simulink model "UAM_Hexa_PD_Obs_QGround"  (R2026a)
settings: Solver=ode4  StopTime=tf  FixedStep=0.01  EnableMultiTasking=on
values from neighbouring files (symbols this model uses):
  ArmConstants = struct('l1_dim', l1_dim,                        'l2_dim', l2_dim,                        'Hexa_to_joint_L', L,                        'Mass1', ml1,                        'Mass2', ml2,                        'Inertia1', Hl1,                        'Inertia2', Hl2,                        'MC1', c1,                        'MC2', c2,                        'Servos', Servos)    [init_model.m]    (also in init_var.m)
  HexaConstants = struct('Mass', mb,                         'Inertia', J ,                         'allo', allo,                          'invallo', invallo,                         'kT', kT)    [init_model.m]    (also in init_var.m)
  Observer = struct('E1', E1 ,     'E2', E2 ,     'E3', E3 ,     'E4', E4 ,     'MU1', MU1 ,     'MU2', MU2 ,     'MU3', MU3 ,     'alpha', alpha ,     'beta', beta)    [init_model.m]    (also in init_var.m)
libraries: px4Utilslib x189
(part 1 of 2)
settings Model: ExtModeTrigDuration=10  Creator=Carlos Fabian  LastModifiedBy=Carlos Fabian
settings SolverCC: PositivePriorityOrder=on
settings HardwareCC: ProdLargestAtomicInteger=Long  ProdLargestAtomicFloat=Double  ProdHWDeviceType=ARM Compatible->ARM Cortex
settings SFSimCC: SimTargetLang=C++
settings RTWCC: SystemTargetFile=ert.tlc  HardwareBoard=PX4 Pixhawk 6c  TLCOptions="-aInlineSetEventsForThisBaseRateFcn=TLC_FALSE -aSuppressMultiTaskScheduler=TLC_FALSE  -aRateBasedStepFcn=0"  Toolchain=GNU Tools for PX4 Autopilots  TargetLang=C++  Description=Embedded Coder
settings ERTTargetCC: ExtModeTransport=3.0  ExtModeStaticAllocSize=1024.0  SupportContinuousTime=on
settings ExplorerConfigSet: InternalSimMechanicsExplorerSettings=|
  | <ExplorerConfiguration>
  | 
  |   <canonicalview>default</canonicalview>
  | 
  |   <TilePanel>
  |     <TileInfo>
  |       <Tiles Columns="1" Count="1" Height="513" Rows="1" Width="774">
  |         <Row Weight="1"/>
  |         <Column Weight="1"/>
  |         <Tile Height="1" Width="1" X="0" Y="0"/>
  |       </Tiles>
  |     </TileInfo>
  |     <SceneInfo>
  |       <SceneViewer>
  |         <IsThisViewStd>
  |           <IsStandardView>off</IsStandardView>
  |           <StandardViewName>Front</StandardViewName>
  |         </IsThisViewStd>
  |         <BGColor>
  |           <R>1</R>
  |           <G>1</G>
  |           <B>1</B>
  |           <A>1</A>
  |         </BGColor>
  |         <Camera>
  |           <DoPerspective>off</DoPerspective>
  |           <Position>
  |             <X>16.201091586104312</X>
  |             <Y>-16.65504514146788</Y>
  |             <Z>17.087073385082522</Z>
  |           </Position>
  |           <Center>
  |             <X>-0.25720946651222221</X>
  |             <Y>-0.19674408885134653</Y>
  |             <Z>0.62877233246599318</Z>
  |           </Center>
  |           <Up>
  |             <X>-0.40824829046386302</X>
  |             <Y>0.40824829046386302</Y>
  |             <Z>0.81649658092772615</Z>
  |           </Up>
  |           <XLim>2.5491252053936631</XLim>
  |           <YLim>2.5491252053936631</YLim>
  |           <ViewLimDist>0.01</ViewLimDist>
  |         </Camera>
  |       </SceneViewer>
  |     </SceneInfo>
  |   </TilePanel>
  | 
  |   <MechEditorPanel>
  |     <GfxPanelCameraMap/>
  |     <Cameras/>
  |     <VideoCreator>
  |       <IncludeTiles>All</IncludeTiles>
  |       <IncludeTime>on</IncludeTime>
  |       <IncludeWorldFrame>off</IncludeWorldFrame>
  |       <PlaybackSpeedRatio>8</PlaybackSpeedRatio>
  |       <FrameRate>24</FrameRate>
  |       <FrameSize>auto</FrameSize>
  |       <VideoFormat>MotionJPEGAVI</VideoFormat>
  |     </VideoCreator>
  |   </MechEditorPanel>
  | 
  |   <PlaybackSettings>
  |     <PlaybackSpeedFactor>16</PlaybackSpeedFactor>
  |   </PlaybackSettings>
  | 
  | </ExplorerConfiguration>

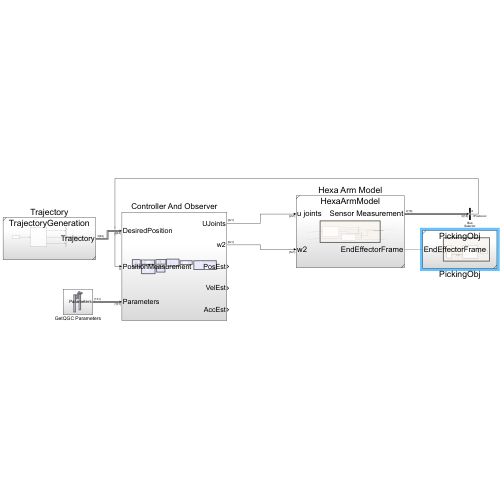
[thumbnail: Simulink's stored preview of the top-level diagram]
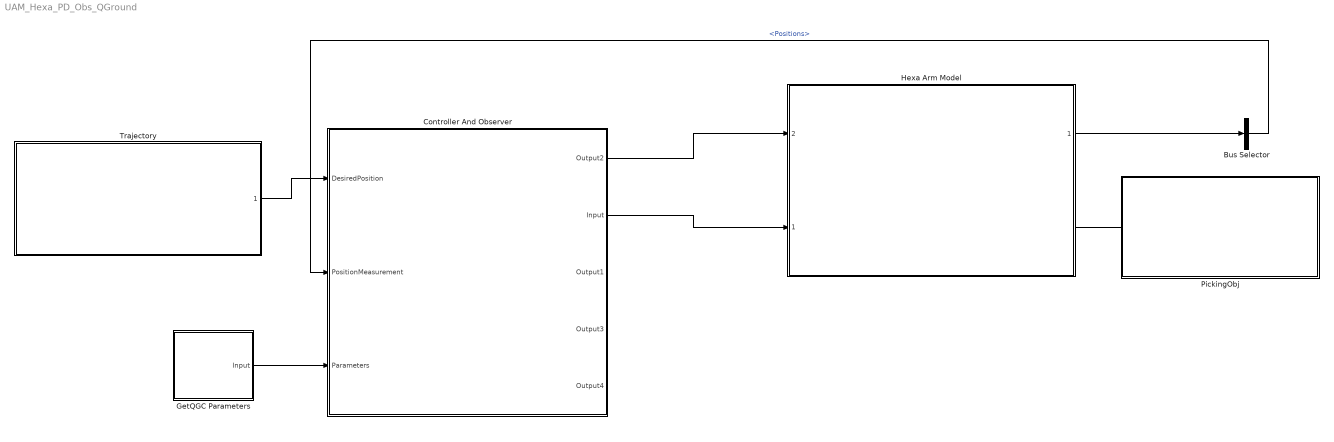
== system UAM_Hexa_PD_Obs_QGround ==
  Bus Selector : BusSelector  OutputSignals=Positions
  Controller And Observer : Subsystem
  GetQGC Parameters : Subsystem
  Hexa Arm Model : Subsystem  ReferencedSubsystem=HexaArmModel
      settings: PortSchema="{\"entries\":[{\"content\":{\"sides\":[{\"content\":{\"connectorIds\":[\"In2\",\"In1\"]},\"type\":\"ConnectorPlacement.EquallySpacedRectSide\",\"uuid\":\"8c321911-c61a-4c60-b031-eeaf4c8b5083\"},{\"content\":{\"connectorIds\":[\"Out1\",\"RConn1\"],\"side\":\"RIGHT\"},\"type\":\"ConnectorPlacement.EquallySpacedRectSide\",\"uuid\":\"3ad1588f-e2f8-4666-8b86-318f5207193d\"},{\"content\":{\"side\":\"TOP\"},\"type\":\"ConnectorPlacement.EquallySpacedRectSide\",\"uuid\":\"710cc49c-59c4-4f69-a558-4588d1d119c0\"}]},\"type\":\"ConnectorPlacement.EquallySpacedConnector\",\"uuid\":\"3e8cca1f-f7f1-4f31-9eba-ef93ff8e81e8\"}],\"packageUris\":[\"http://schema.mathworks.com/mf0/Connector/R2020b\"],\"version\":\"1.0\"}"
  PickingObj : Subsystem  ReferencedSubsystem=PickingObj
  Trajectory : Subsystem  ReferencedSubsystem=TrajectoryGeneration
  wires:
  Controller And Observer/2(Input) -> Hexa Arm Model/1
  Trajectory/1 -> Controller And Observer/1(DesiredPosition)
  Hexa Arm Model/1 -> Bus Selector/1
  Controller And Observer/1(Output2) -> Hexa Arm Model/2
  Bus Selector/1 -> Controller And Observer/2(PositionMeasurement)  "<Positions>"
  GetQGC Parameters/1(Input) -> Controller And Observer/3(Parameters)
  connections:
  Hexa Arm Model/RConn1 -- PickingObj/LConn1

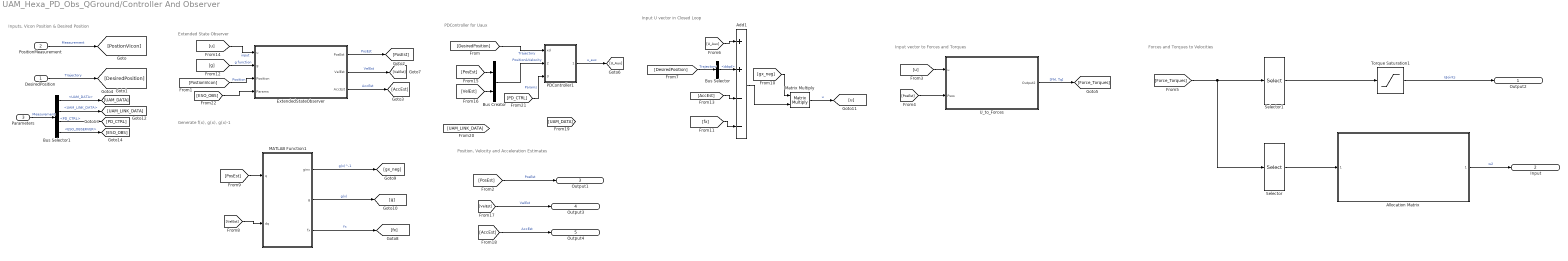
== system UAM_Hexa_PD_Obs_QGround/Controller And Observer ==
  note: Position, Velocity and Acceleration Estimates
  note: Input vector to Forces and Torques
  note: Forces and Torques to Velocities
  note: Extended State Observer
  note: Input U vector in Closed Loop
  note: Generate f(x), g(x), g(x)-1
  note: PDController for Uaux
  note: Inputs, Vicon Position & Desired Position
  DesiredPosition : Inport  SampleTime=0.01
  PositionMeasurement : Inport  Port=2  SampleTime=0.01
  Parameters : Inport  Port=3  SampleTime=0.01
  Add1 : Sum  Inputs=++--
  Allocation Matrix : Subsystem  ReferencedSubsystem=FromFMtoOmega2
  Bus Creator : BusCreator  Inputs=2
  Bus Selector : BusSelector  OutputSignals=ddqd
  Bus Selector1 : BusSelector  OutputSignals=UAM_DATA,UAM_LINK_DATA,PD_CTRL,ESO_OBSERVER
  ExtendedStateObserver : Subsystem
  MATLAB Function1 : MATLAB Function  TreatAsAtomicUnit=on
  Matrix Multiply : Product  Multiplication=Matrix(*)
  PDController1 : Subsystem
  Selector : Selector  InputPortWidth=8  IndexOptions=Index vector (dialog)  Indices=1:6  OutputSizes=1
  Selector1 : Selector  InputPortWidth=8  IndexOptions=Index vector (dialog)  Indices=7:8  OutputSizes=1
  Torque Saturation1 : Saturate  UpperLimit=ArmConstants.Servos.T1max  LowerLimit=-ArmConstants.Servos.T1max
  U_to_Forces : Subsystem
  Output2 : Outport  SampleTime=0.01
  Input : Outport  Port=2  SampleTime=0.01
  Output1 : Outport  Port=3  SampleTime=0.01
  Output3 : Outport  Port=4  SampleTime=0.01
  Output4 : Outport  Port=5  SampleTime=0.01
  wires:
  [PostionVicon] -> ExtendedStateObserver/3(Position)  "Position"
  [DesiredPosition] -> PDController1/1(xd)  "Trajectory"
  U_to_Forces/1(Output2) -> [Force_Torques]  "[FM, Tq]"
  ExtendedStateObserver/1(PosEst) -> [PosEst]  "PosEst"
  PositionMeasurement/1 -> [PostionVicon]  "Measurement"
  DesiredPosition/1 -> [DesiredPosition]  "Trajectory"
  Bus Creator/1 -> PDController1/2(q_hat1)  "Position&Velocity"
  ExtendedStateObserver/3(AccEst) -> [AccEst]  "AccEst"
  ExtendedStateObserver/2(VelEst) -> [VelEst]  "VelEst"
  [PosEst] -> U_to_Forces/2(Psos)
  Selector1/1 -> Torque Saturation1/1
  [Force_Torques] -> Selector/1, Selector1/1
  Selector/1 -> Allocation Matrix/1
  Torque Saturation1/1 -> Output2/1  "UJoints"
  Allocation Matrix/1 -> Input/1  "w2"
  PDController1/1(Output) -> [U_Aux]  "u_aux"
  MATLAB Function1/1(ginv) -> [gx_neg]  "g(x)^-1"
  MATLAB Function1/3(fx) -> [fx]  "fx"
  [VelEst] -> MATLAB Function1/2(dq)
  [PosEst] -> MATLAB Function1/1(q)
  [fx] -> Add1/4
  Add1/1 -> Matrix Multiply/2
  Matrix Multiply/1 -> [u]  "u"
  [gx_neg] -> Matrix Multiply/1
  [U_Aux] -> Add1/1
  [DesiredPosition] -> Bus Selector/1  "Trajectory"
  Bus Selector/1 -> Add1/2  "<ddqd>"
  [AccEst] -> Add1/3
  MATLAB Function1/2(g) -> [g]  "g(x)"
  [g] -> ExtendedStateObserver/2(g)  "g function"
  [u] -> ExtendedStateObserver/1(u)  "input"
  [PosEst] -> Bus Creator/1
  [VelEst] -> Bus Creator/2
  [u] -> U_to_Forces/1(u)
  [PosEst] -> Output1/1  "PosEst"
  [VelEst] -> Output3/1  "VelEst"
  [AccEst] -> Output4/1  "AccEst"
  Parameters/1 -> Bus Selector1/1  "Measurement"
  Bus Selector1/1 -> [UAM_DATA]  "<UAM_DATA>"
  Bus Selector1/4 -> [ESO_OBS]  "<ESO_OBSERVER>"
  Bus Selector1/3 -> [PD_CTRL]  "<PD_CTRL>"
  Bus Selector1/2 -> [UAM_LINK_DATA]  "<UAM_LINK_DATA>"
  [ESO_OBS] -> ExtendedStateObserver/4(Params)
  [PD_CTRL] -> PDController1/3(Params)  "Params"

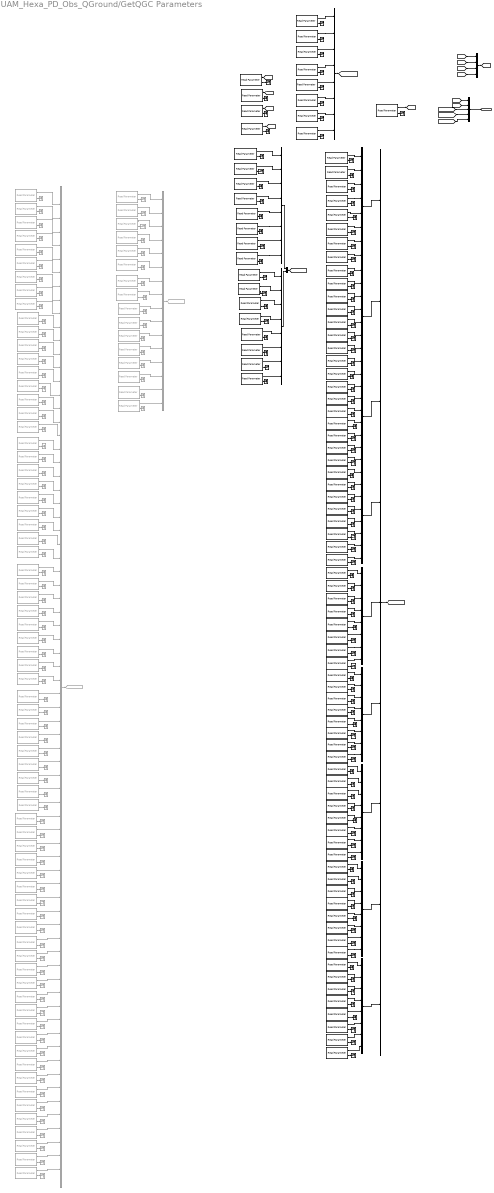
== system UAM_Hexa_PD_Obs_QGround/GetQGC Parameters ==
  note: Create Parameters Bus
  note: Parameter Manipulator
  note: Parameters FAH
  note: Parameter PD controller
  note: Parameter ESO
  note: Parameter Manipulator
  note: Parameter PD controller
  note: Parameter ESO
  Bus Creator : BusCreator  Inputs=5
  Bus Creator1 : BusCreator  Inputs=4
  Bus Creator2 : BusCreator  Inputs=2
  Bus Creator3 : BusCreator  Inputs=8
  Bus Creator4 : BusCreator  Inputs=9
  Bus Creator5 : BusCreator  Commented=on  Inputs=16
  Bus Creator6 : BusCreator  Commented=on  Inputs=72
  Goto10 : Goto  Commented=on  GotoTag=ESO_OBSERVER
  Goto9 : Goto  Commented=on  GotoTag=PD_CTRL
  Mux{,1..10} (11 alike) : Mux  Inputs=8
  Read Parameter1 : px4Utilslib/Read Parameter  ParameterName=UAM_MASS  DataType=FLOAT  SampleTime=inf
  Read Parameter10 : px4Utilslib/Read Parameter  ParameterName=UAM_L_ONE_I_ZZ  DataType=FLOAT  SampleTime=inf
  Read Parameter100 : px4Utilslib/Read Parameter  ParameterName=L_TWO_E1  DataType=FLOAT  SampleTime=inf
  Read Parameter101 : px4Utilslib/Read Parameter  ParameterName=TRAJ_SEL  DataType=INT32  SampleTime=inf
  Read Parameter102 : px4Utilslib/Read Parameter  Commented=on  ParameterName=UAM_X_P  DataType=FLOAT  SampleTime=inf
  Read Parameter103 : px4Utilslib/Read Parameter  Commented=on  ParameterName=UAM_Y_P  DataType=FLOAT  SampleTime=inf
  Read Parameter104 : px4Utilslib/Read Parameter  Commented=on  ParameterName=UAM_Y_D  DataType=FLOAT  SampleTime=inf
  Read Parameter105 : px4Utilslib/Read Parameter  Commented=on  ParameterName=UAM_Z_P  DataType=FLOAT  SampleTime=inf
  Read Parameter106 : px4Utilslib/Read Parameter  Commented=on  ParameterName=UAM_Z_D  DataType=FLOAT  SampleTime=inf
  Read Parameter107 : px4Utilslib/Read Parameter  Commented=on  ParameterName=UAM_ROLL_P  DataType=FLOAT  SampleTime=inf
  Read Parameter108 : px4Utilslib/Read Parameter  Commented=on  ParameterName=UAM_PITCH_P  DataType=FLOAT  SampleTime=inf
  Read Parameter109 : px4Utilslib/Read Parameter  Commented=on  ParameterName=UAM_PITCH_D  DataType=FLOAT  SampleTime=inf
  Read Parameter11 : px4Utilslib/Read Parameter  ParameterName=UAM_L_TWO_I_ZZ  DataType=FLOAT  SampleTime=inf
  Read Parameter110 : px4Utilslib/Read Parameter  Commented=on  ParameterName=UAM_YAW_P  DataType=FLOAT  SampleTime=inf
  Read Parameter111 : px4Utilslib/Read Parameter  Commented=on  ParameterName=UAM_YAW_D  DataType=FLOAT  SampleTime=inf
  Read Parameter112 : px4Utilslib/Read Parameter  Commented=on  ParameterName=UAM_ROLL_D  DataType=FLOAT  SampleTime=inf
  Read Parameter113 : px4Utilslib/Read Parameter  Commented=on  ParameterName=UAM_L_ONE_P  DataType=FLOAT  SampleTime=inf
  Read Parameter114 : px4Utilslib/Read Parameter  Commented=on  ParameterName=UAM_L_ONE_D  DataType=FLOAT  SampleTime=inf
  Read Parameter115 : px4Utilslib/Read Parameter  Commented=on  ParameterName=UAM_L_TWO_P  DataType=FLOAT  SampleTime=inf
  Read Parameter116 : px4Utilslib/Read Parameter  Commented=on  ParameterName=UAM_L_TWO_D  DataType=FLOAT  SampleTime=inf
  Read Parameter117 : px4Utilslib/Read Parameter  Commented=on  ParameterName=UAM_X_D  DataType=FLOAT  SampleTime=inf
  Read Parameter118 : px4Utilslib/Read Parameter  Commented=on  ParameterName=L_TWO_E1  DataType=FLOAT  SampleTime=inf
  Read Parameter119 : px4Utilslib/Read Parameter  Commented=on  ParameterName=X_E2  DataType=FLOAT  SampleTime=inf
  Read Parameter12 : px4Utilslib/Read Parameter  ParameterName=UAM_L_TWO_MASS  DataType=FLOAT  SampleTime=inf
  Read Parameter120 : px4Utilslib/Read Parameter  Commented=on  ParameterName=X_E3  DataType=FLOAT  SampleTime=inf
  Read Parameter121 : px4Utilslib/Read Parameter  Commented=on  ParameterName=X_E4  DataType=FLOAT  SampleTime=inf
  Read Parameter122 : px4Utilslib/Read Parameter  Commented=on  ParameterName=X_MU2  DataType=FLOAT  SampleTime=inf
  Read Parameter123 : px4Utilslib/Read Parameter  Commented=on  ParameterName=X_MU3  DataType=FLOAT  SampleTime=inf
  Read Parameter124 : px4Utilslib/Read Parameter  Commented=on  ParameterName=X_MU1  DataType=FLOAT  SampleTime=inf
  Read Parameter125 : px4Utilslib/Read Parameter  Commented=on  ParameterName=X_BETA  DataType=FLOAT  SampleTime=inf
  Read Parameter126 : px4Utilslib/Read Parameter  Commented=on  ParameterName=X_ALPHA  DataType=FLOAT  SampleTime=inf
  Read Parameter127 : px4Utilslib/Read Parameter  Commented=on  ParameterName=Y_E2  DataType=FLOAT  SampleTime=inf
  Read Parameter128 : px4Utilslib/Read Parameter  Commented=on  ParameterName=Y_E3  DataType=FLOAT  SampleTime=inf
  Read Parameter129 : px4Utilslib/Read Parameter  Commented=on  ParameterName=X_E1  DataType=FLOAT  SampleTime=inf
  Read Parameter13 : px4Utilslib/Read Parameter  ParameterName=UAM_L_TWO_I_XX  DataType=FLOAT  SampleTime=inf
  Read Parameter130 : px4Utilslib/Read Parameter  Commented=on  ParameterName=Y_E4  DataType=FLOAT  SampleTime=inf
  Read Parameter131 : px4Utilslib/Read Parameter  Commented=on  ParameterName=Y_MU2  DataType=FLOAT  SampleTime=inf
  Read Parameter132 : px4Utilslib/Read Parameter  Commented=on  ParameterName=Y_MU3  DataType=FLOAT  SampleTime=inf
  Read Parameter133 : px4Utilslib/Read Parameter  Commented=on  ParameterName=Y_MU1  DataType=FLOAT  SampleTime=inf
  Read Parameter134 : px4Utilslib/Read Parameter  Commented=on  ParameterName=Y_BETA  DataType=FLOAT  SampleTime=inf
  Read Parameter135 : px4Utilslib/Read Parameter  Commented=on  ParameterName=Y_ALPHA  DataType=FLOAT  SampleTime=inf
  Read Parameter136 : px4Utilslib/Read Parameter  Commented=on  ParameterName=Y_E1  DataType=FLOAT  SampleTime=inf
  Read Parameter137 : px4Utilslib/Read Parameter  Commented=on  ParameterName=Z_E2  DataType=FLOAT  SampleTime=inf
  Read Parameter138 : px4Utilslib/Read Parameter  Commented=on  ParameterName=Z_E3  DataType=FLOAT  SampleTime=inf
  Read Parameter139 : px4Utilslib/Read Parameter  Commented=on  ParameterName=Z_E4  DataType=FLOAT  SampleTime=inf
  Read Parameter14 : px4Utilslib/Read Parameter  ParameterName=UAM_L_TWO_I_YY  DataType=FLOAT  SampleTime=inf
  Read Parameter140 : px4Utilslib/Read Parameter  Commented=on  ParameterName=Z_MU2  DataType=FLOAT  SampleTime=inf
  Read Parameter141 : px4Utilslib/Read Parameter  Commented=on  ParameterName=Z_MU3  DataType=FLOAT  SampleTime=inf
  Read Parameter142 : px4Utilslib/Read Parameter  Commented=on  ParameterName=Z_MU1  DataType=FLOAT  SampleTime=inf
  Read Parameter143 : px4Utilslib/Read Parameter  Commented=on  ParameterName=Z_BETA  DataType=FLOAT  SampleTime=inf
  Read Parameter144 : px4Utilslib/Read Parameter  Commented=on  ParameterName=Z_ALPHA  DataType=FLOAT  SampleTime=inf
  Read Parameter145 : px4Utilslib/Read Parameter  Commented=on  ParameterName=Z_E1  DataType=FLOAT  SampleTime=inf
  Read Parameter146 : px4Utilslib/Read Parameter  Commented=on  ParameterName=ROLL_E2  DataType=FLOAT  SampleTime=inf
  Read Parameter147 : px4Utilslib/Read Parameter  Commented=on  ParameterName=ROLL_E3  DataType=FLOAT  SampleTime=inf
  Read Parameter148 : px4Utilslib/Read Parameter  Commented=on  ParameterName=ROLL_E4  DataType=FLOAT  SampleTime=inf
  Read Parameter149 : px4Utilslib/Read Parameter  Commented=on  ParameterName=ROLL_MU2  DataType=FLOAT  SampleTime=inf
  Read Parameter15 : px4Utilslib/Read Parameter  ParameterName=UAM_X_P  DataType=FLOAT  SampleTime=inf
  Read Parameter150 : px4Utilslib/Read Parameter  Commented=on  ParameterName=ROLL_MU3  DataType=FLOAT  SampleTime=inf
  Read Parameter151 : px4Utilslib/Read Parameter  Commented=on  ParameterName=ROLL_MU1  DataType=FLOAT  SampleTime=inf
  Read Parameter152 : px4Utilslib/Read Parameter  Commented=on  ParameterName=ROLL_BETA  DataType=FLOAT  SampleTime=inf
  Read Parameter153 : px4Utilslib/Read Parameter  Commented=on  ParameterName=ROLL_ALPHA  DataType=FLOAT  SampleTime=inf
  Read Parameter154 : px4Utilslib/Read Parameter  Commented=on  ParameterName=ROLL_E1  DataType=FLOAT  SampleTime=inf
  Read Parameter155 : px4Utilslib/Read Parameter  Commented=on  ParameterName=PITCH_E2  DataType=FLOAT  SampleTime=inf
  Read Parameter156 : px4Utilslib/Read Parameter  Commented=on  ParameterName=PITCH_E3  DataType=FLOAT  SampleTime=inf
  Read Parameter157 : px4Utilslib/Read Parameter  Commented=on  ParameterName=PITCH_E4  DataType=FLOAT  SampleTime=inf
  Read Parameter158 : px4Utilslib/Read Parameter  Commented=on  ParameterName=PITCH_MU2  DataType=FLOAT  SampleTime=inf
  Read Parameter159 : px4Utilslib/Read Parameter  Commented=on  ParameterName=PITCH_MU3  DataType=FLOAT  SampleTime=inf
  Read Parameter16 : px4Utilslib/Read Parameter  ParameterName=UAM_Y_P  DataType=FLOAT  SampleTime=inf
  Read Parameter160 : px4Utilslib/Read Parameter  Commented=on  ParameterName=PITCH_MU1  DataType=FLOAT  SampleTime=inf
  Read Parameter161 : px4Utilslib/Read Parameter  Commented=on  ParameterName=PITCH_BETA  DataType=FLOAT  SampleTime=inf
  Read Parameter162 : px4Utilslib/Read Parameter  Commented=on  ParameterName=PITCH_ALPHA  DataType=FLOAT  SampleTime=inf
  Read Parameter163 : px4Utilslib/Read Parameter  Commented=on  ParameterName=PITCH_E1  DataType=FLOAT  SampleTime=inf
  Read Parameter164 : px4Utilslib/Read Parameter  Commented=on  ParameterName=YAW_E2  DataType=FLOAT  SampleTime=inf
  Read Parameter165 : px4Utilslib/Read Parameter  Commented=on  ParameterName=YAW_E3  DataType=FLOAT  SampleTime=inf
  Read Parameter166 : px4Utilslib/Read Parameter  Commented=on  ParameterName=YAW_E4  DataType=FLOAT  SampleTime=inf
  Read Parameter167 : px4Utilslib/Read Parameter  Commented=on  ParameterName=YAW_MU2  DataType=FLOAT  SampleTime=inf
  Read Parameter168 : px4Utilslib/Read Parameter  Commented=on  ParameterName=YAW_MU3  DataType=FLOAT  SampleTime=inf
  Read Parameter169 : px4Utilslib/Read Parameter  Commented=on  ParameterName=YAW_MU1  DataType=FLOAT  SampleTime=inf
  Read Parameter17 : px4Utilslib/Read Parameter  ParameterName=UAM_Y_D  DataType=FLOAT  SampleTime=inf
  Read Parameter170 : px4Utilslib/Read Parameter  Commented=on  ParameterName=YAW_BETA  DataType=FLOAT  SampleTime=inf
  Read Parameter171 : px4Utilslib/Read Parameter  Commented=on  ParameterName=YAW_ALPHA  DataType=FLOAT  SampleTime=inf
  Read Parameter172 : px4Utilslib/Read Parameter  Commented=on  ParameterName=YAW_E1  DataType=FLOAT  SampleTime=inf
  Read Parameter173 : px4Utilslib/Read Parameter  Commented=on  ParameterName=L_ONE_E2  DataType=FLOAT  SampleTime=inf
  Read Parameter174 : px4Utilslib/Read Parameter  Commented=on  ParameterName=L_ONE_E3  DataType=FLOAT  SampleTime=inf
  Read Parameter175 : px4Utilslib/Read Parameter  Commented=on  ParameterName=L_ONE_E4  DataType=FLOAT  SampleTime=inf
  Read Parameter176 : px4Utilslib/Read Parameter  Commented=on  ParameterName=L_ONE_MU2  DataType=FLOAT  SampleTime=inf
  Read Parameter177 : px4Utilslib/Read Parameter  Commented=on  ParameterName=L_ONE_MU3  DataType=FLOAT  SampleTime=inf
  Read Parameter178 : px4Utilslib/Read Parameter  Commented=on  ParameterName=L_ONE_MU1  DataType=FLOAT  SampleTime=inf
  Read Parameter179 : px4Utilslib/Read Parameter  Commented=on  ParameterName=L_ONE_BETA  DataType=FLOAT  SampleTime=inf
  Read Parameter18 : px4Utilslib/Read Parameter  ParameterName=UAM_Z_P  DataType=FLOAT  SampleTime=inf
  Read Parameter180 : px4Utilslib/Read Parameter  Commented=on  ParameterName=L_ONE_ALPHA  DataType=FLOAT  SampleTime=inf
  Read Parameter181 : px4Utilslib/Read Parameter  Commented=on  ParameterName=L_TWO_E2  DataType=FLOAT  SampleTime=inf
  Read Parameter182 : px4Utilslib/Read Parameter  Commented=on  ParameterName=L_TWO_E3  DataType=FLOAT  SampleTime=inf
  Read Parameter183 : px4Utilslib/Read Parameter  Commented=on  ParameterName=L_ONE_E1  DataType=FLOAT  SampleTime=inf
  Read Parameter184 : px4Utilslib/Read Parameter  Commented=on  ParameterName=L_TWO_E4  DataType=FLOAT  SampleTime=inf
  Read Parameter185 : px4Utilslib/Read Parameter  Commented=on  ParameterName=L_TWO_MU2  DataType=FLOAT  SampleTime=inf
  Read Parameter186 : px4Utilslib/Read Parameter  Commented=on  ParameterName=L_TWO_MU3  DataType=FLOAT  SampleTime=inf
  Read Parameter187 : px4Utilslib/Read Parameter  Commented=on  ParameterName=L_TWO_MU1  DataType=FLOAT  SampleTime=inf
  Read Parameter188 : px4Utilslib/Read Parameter  Commented=on  ParameterName=L_TWO_BETA  DataType=FLOAT  SampleTime=inf
  Read Parameter189 : px4Utilslib/Read Parameter  Commented=on  ParameterName=L_TWO_ALPHA  DataType=FLOAT  SampleTime=inf
  Read Parameter19 : px4Utilslib/Read Parameter  ParameterName=UAM_Z_D  DataType=FLOAT  SampleTime=inf
  Read Parameter2 : px4Utilslib/Read Parameter  ParameterName=UAM_L_ONE_MASS  DataType=FLOAT  SampleTime=inf
  Read Parameter20 : px4Utilslib/Read Parameter  ParameterName=UAM_ROLL_P  DataType=FLOAT  SampleTime=inf
  Read Parameter21 : px4Utilslib/Read Parameter  ParameterName=UAM_PITCH_P  DataType=FLOAT  SampleTime=inf
  Read Parameter22 : px4Utilslib/Read Parameter  ParameterName=UAM_PITCH_D  DataType=FLOAT  SampleTime=inf
  Read Parameter23 : px4Utilslib/Read Parameter  ParameterName=UAM_YAW_P  DataType=FLOAT  SampleTime=inf
  Read Parameter24 : px4Utilslib/Read Parameter  ParameterName=UAM_YAW_D  DataType=FLOAT  SampleTime=inf
  Read Parameter25 : px4Utilslib/Read Parameter  ParameterName=UAM_ROLL_D  DataType=FLOAT  SampleTime=inf
  Read Parameter26 : px4Utilslib/Read Parameter  ParameterName=UAM_L_ONE_P  DataType=FLOAT  SampleTime=inf
  Read Parameter27 : px4Utilslib/Read Parameter  ParameterName=UAM_L_ONE_D  DataType=FLOAT  SampleTime=inf
  Read Parameter28 : px4Utilslib/Read Parameter  ParameterName=UAM_L_TWO_P  DataType=FLOAT  SampleTime=inf
  Read Parameter29 : px4Utilslib/Read Parameter  ParameterName=UAM_L_TWO_D  DataType=FLOAT  SampleTime=inf
  Read Parameter3 : px4Utilslib/Read Parameter  ParameterName=UAM_X_D  DataType=FLOAT  SampleTime=inf
  Read Parameter30 : px4Utilslib/Read Parameter  ParameterName=X_E2  DataType=FLOAT  SampleTime=inf
  Read Parameter31 : px4Utilslib/Read Parameter  ParameterName=X_E3  DataType=FLOAT  SampleTime=inf
  Read Parameter32 : px4Utilslib/Read Parameter  ParameterName=X_E4  DataType=FLOAT  SampleTime=inf
  Read Parameter33 : px4Utilslib/Read Parameter  ParameterName=X_MU2  DataType=FLOAT  SampleTime=inf
  Read Parameter34 : px4Utilslib/Read Parameter  ParameterName=X_MU3  DataType=FLOAT  SampleTime=inf
  Read Parameter35 : px4Utilslib/Read Parameter  ParameterName=X_MU1  DataType=FLOAT  SampleTime=inf
  Read Parameter36 : px4Utilslib/Read Parameter  ParameterName=X_BETA  DataType=FLOAT  SampleTime=inf
  Read Parameter37 : px4Utilslib/Read Parameter  ParameterName=X_ALPHA  DataType=FLOAT  SampleTime=inf
  Read Parameter38 : px4Utilslib/Read Parameter  ParameterName=Y_E2  DataType=FLOAT  SampleTime=inf
  Read Parameter39 : px4Utilslib/Read Parameter  ParameterName=Y_E3  DataType=FLOAT  SampleTime=inf
  Read Parameter4 : px4Utilslib/Read Parameter  ParameterName=X_E1  DataType=FLOAT  SampleTime=inf
  Read Parameter40 : px4Utilslib/Read Parameter  ParameterName=Y_E4  DataType=FLOAT  SampleTime=inf
  Read Parameter41 : px4Utilslib/Read Parameter  ParameterName=Y_MU2  DataType=FLOAT  SampleTime=inf
  Read Parameter42 : px4Utilslib/Read Parameter  ParameterName=Y_MU3  DataType=FLOAT  SampleTime=inf
  Read Parameter43 : px4Utilslib/Read Parameter  ParameterName=Y_MU1  DataType=FLOAT  SampleTime=inf
  Read Parameter44 : px4Utilslib/Read Parameter  ParameterName=Y_BETA  DataType=FLOAT  SampleTime=inf
  Read Parameter45 : px4Utilslib/Read Parameter  ParameterName=Y_ALPHA  DataType=FLOAT  SampleTime=inf
  Read Parameter46 : px4Utilslib/Read Parameter  ParameterName=Y_E1  DataType=FLOAT  SampleTime=inf
  Read Parameter47 : px4Utilslib/Read Parameter  ParameterName=Z_E2  DataType=FLOAT  SampleTime=inf
  Read Parameter48 : px4Utilslib/Read Parameter  ParameterName=Z_E3  DataType=FLOAT  SampleTime=inf
  Read Parameter49 : px4Utilslib/Read Parameter  ParameterName=Z_E4  DataType=FLOAT  SampleTime=inf
  Read Parameter5 : px4Utilslib/Read Parameter  ParameterName=UAM_I_XX  DataType=FLOAT  SampleTime=inf
  Read Parameter50 : px4Utilslib/Read Parameter  ParameterName=Z_MU2  DataType=FLOAT  SampleTime=inf
  Read Parameter51 : px4Utilslib/Read Parameter  ParameterName=Z_MU3  DataType=FLOAT  SampleTime=inf
  Read Parameter52 : px4Utilslib/Read Parameter  ParameterName=Z_MU1  DataType=FLOAT  SampleTime=inf
  Read Parameter53 : px4Utilslib/Read Parameter  ParameterName=Z_BETA  DataType=FLOAT  SampleTime=inf
  Read Parameter54 : px4Utilslib/Read Parameter  ParameterName=Z_ALPHA  DataType=FLOAT  SampleTime=inf
  Read Parameter55 : px4Utilslib/Read Parameter  ParameterName=Z_E1  DataType=FLOAT  SampleTime=inf
  Read Parameter56 : px4Utilslib/Read Parameter  ParameterName=ROLL_E2  DataType=FLOAT  SampleTime=inf
  Read Parameter57 : px4Utilslib/Read Parameter  ParameterName=ROLL_E3  DataType=FLOAT  SampleTime=inf
  Read Parameter58 : px4Utilslib/Read Parameter  ParameterName=ROLL_E4  DataType=FLOAT  SampleTime=inf
  Read Parameter59 : px4Utilslib/Read Parameter  ParameterName=ROLL_MU2  DataType=FLOAT  SampleTime=inf
  Read Parameter6 : px4Utilslib/Read Parameter  ParameterName=UAM_I_YY  DataType=FLOAT  SampleTime=inf
  Read Parameter60 : px4Utilslib/Read Parameter  ParameterName=ROLL_MU3  DataType=FLOAT  SampleTime=inf
  Read Parameter61 : px4Utilslib/Read Parameter  ParameterName=ROLL_MU1  DataType=FLOAT  SampleTime=inf
  Read Parameter62 : px4Utilslib/Read Parameter  ParameterName=ROLL_BETA  DataType=FLOAT  SampleTime=inf
  Read Parameter63 : px4Utilslib/Read Parameter  ParameterName=ROLL_ALPHA  DataType=FLOAT  SampleTime=inf
  Read Parameter64 : px4Utilslib/Read Parameter  ParameterName=ROLL_E1  DataType=FLOAT  SampleTime=inf
  Read Parameter65 : px4Utilslib/Read Parameter  ParameterName=PITCH_E2  DataType=FLOAT  SampleTime=inf
  Read Parameter66 : px4Utilslib/Read Parameter  ParameterName=PITCH_E3  DataType=FLOAT  SampleTime=inf
  Read Parameter67 : px4Utilslib/Read Parameter  ParameterName=PITCH_E4  DataType=FLOAT  SampleTime=inf
  Read Parameter68 : px4Utilslib/Read Parameter  ParameterName=PITCH_MU2  DataType=FLOAT  SampleTime=inf
  Read Parameter69 : px4Utilslib/Read Parameter  ParameterName=PITCH_MU3  DataType=FLOAT  SampleTime=inf
  Read Parameter7 : px4Utilslib/Read Parameter  ParameterName=UAM_I_ZZ  DataType=FLOAT  SampleTime=inf
  Read Parameter70 : px4Utilslib/Read Parameter  ParameterName=PITCH_MU1  DataType=FLOAT  SampleTime=inf
  Read Parameter71 : px4Utilslib/Read Parameter  ParameterName=PITCH_BETA  DataType=FLOAT  SampleTime=inf
  Read Parameter72 : px4Utilslib/Read Parameter  ParameterName=PITCH_ALPHA  DataType=FLOAT  SampleTime=inf
  Read Parameter73 : px4Utilslib/Read Parameter  ParameterName=PITCH_E1  DataType=FLOAT  SampleTime=inf
  Read Parameter74 : px4Utilslib/Read Parameter  ParameterName=YAW_E2  DataType=FLOAT  SampleTime=inf
  Read Parameter75 : px4Utilslib/Read Parameter  ParameterName=YAW_E3  DataType=FLOAT  SampleTime=inf
  Read Parameter76 : px4Utilslib/Read Parameter  ParameterName=YAW_E4  DataType=FLOAT  SampleTime=inf
  Read Parameter77 : px4Utilslib/Read Parameter  ParameterName=YAW_MU2  DataType=FLOAT  SampleTime=inf
  Read Parameter78 : px4Utilslib/Read Parameter  ParameterName=YAW_MU3  DataType=FLOAT  SampleTime=inf
  Read Parameter79 : px4Utilslib/Read Parameter  ParameterName=YAW_MU1  DataType=FLOAT  SampleTime=inf
  Read Parameter8 : px4Utilslib/Read Parameter  ParameterName=UAM_L_ONE_I_XX  DataType=FLOAT  SampleTime=inf
  Read Parameter80 : px4Utilslib/Read Parameter  ParameterName=YAW_BETA  DataType=FLOAT  SampleTime=inf
  Read Parameter81 : px4Utilslib/Read Parameter  ParameterName=YAW_ALPHA  DataType=FLOAT  SampleTime=inf
  Read Parameter82 : px4Utilslib/Read Parameter  ParameterName=YAW_E1  DataType=FLOAT  SampleTime=inf
  Read Parameter83 : px4Utilslib/Read Parameter  ParameterName=L_ONE_E2  DataType=FLOAT  SampleTime=inf
  Read Parameter84 : px4Utilslib/Read Parameter  ParameterName=L_ONE_E3  DataType=FLOAT  SampleTime=inf
  Read Parameter85 : px4Utilslib/Read Parameter  ParameterName=L_ONE_E4  DataType=FLOAT  SampleTime=inf
  Read Parameter86 : px4Utilslib/Read Parameter  ParameterName=L_ONE_MU2  DataType=FLOAT  SampleTime=inf
  Read Parameter87 : px4Utilslib/Read Parameter  ParameterName=L_ONE_MU3  DataType=FLOAT  SampleTime=inf
  Read Parameter88 : px4Utilslib/Read Parameter  ParameterName=L_ONE_MU1  DataType=FLOAT  SampleTime=inf
  Read Parameter89 : px4Utilslib/Read Parameter  ParameterName=L_ONE_BETA  DataType=FLOAT  SampleTime=inf
  Read Parameter9 : px4Utilslib/Read Parameter  ParameterName=UAM_L_ONE_I_YY  DataType=FLOAT  SampleTime=inf
  Read Parameter90 : px4Utilslib/Read Parameter  ParameterName=L_ONE_ALPHA  DataType=FLOAT  SampleTime=inf
  Read Parameter91 : px4Utilslib/Read Parameter  ParameterName=L_TWO_E2  DataType=FLOAT  SampleTime=inf
  Read Parameter92 : px4Utilslib/Read Parameter  ParameterName=L_TWO_E3  DataType=FLOAT  SampleTime=inf
  Read Parameter93 : px4Utilslib/Read Parameter  ParameterName=L_ONE_E1  DataType=FLOAT  SampleTime=inf
  Read Parameter94 : px4Utilslib/Read Parameter  ParameterName=L_TWO_E4  DataType=FLOAT  SampleTime=inf
  Read Parameter95 : px4Utilslib/Read Parameter  ParameterName=L_TWO_MU2  DataType=FLOAT  SampleTime=inf
  Read Parameter96 : px4Utilslib/Read Parameter  ParameterName=L_TWO_MU3  DataType=FLOAT  SampleTime=inf
  Read Parameter97 : px4Utilslib/Read Parameter  ParameterName=L_TWO_MU1  DataType=FLOAT  SampleTime=inf
  Read Parameter98 : px4Utilslib/Read Parameter  ParameterName=L_TWO_BETA  DataType=FLOAT  SampleTime=inf
  Read Parameter99 : px4Utilslib/Read Parameter  ParameterName=L_TWO_ALPHA  DataType=FLOAT  SampleTime=inf
  Terminator{,1..100} (101 alike) : Terminator
  Terminator{101..188} (88 alike) : Terminator  Commented=on
  Input : Outport  SampleTime=0.01
  wires:
  Read Parameter1/2 -> Terminator/1
  Read Parameter1/1 -> [UAM_Mass]
  Read Parameter5/1 -> [UAM_I_XX]
  Read Parameter5/2 -> Terminator1/1
  Read Parameter6/2 -> Terminator2/1
  Read Parameter6/1 -> [UAM_I_YY]
  Read Parameter7/2 -> Terminator3/1
  Read Parameter7/1 -> [UAM_I_ZZ]
  [UAM_Mass] -> Bus Creator1/1  "UAM_MASS"
  Bus Creator/1 -> Input/1  "Parameters"
  Bus Creator1/1 -> [UAM_Data]
  [UAM_I_XX] -> Bus Creator1/2  "UAM_I_XX"
  [UAM_I_YY] -> Bus Creator1/3  "UAM_I_YY"
  [UAM_I_ZZ] -> Bus Creator1/4  "UAM_I_ZZ"
  Read Parameter101/1 -> [TRAJ_SEL]
  Read Parameter101/2 -> Terminator4/1
  [TRAJ_SEL] -> Bus Creator/2  "TRAJ_SEL"
  [UAM_Data] -> Bus Creator/1  "UAM_DATA"
  [PD_CTRL] -> Bus Creator/3  "PD_CTRL"
  Read Parameter15/2 -> Terminator5/1
  Read Parameter3/2 -> Terminator6/1
  Read Parameter16/2 -> Terminator7/1
  Read Parameter17/2 -> Terminator8/1
  Read Parameter18/2 -> Terminator9/1
  Read Parameter19/2 -> Terminator10/1
  Read Parameter26/2 -> Terminator11/1
  Read Parameter27/2 -> Terminator12/1
  Read Parameter20/2 -> Terminator13/1
  Read Parameter25/2 -> Terminator14/1
  Read Parameter21/2 -> Terminator15/1
  Read Parameter22/2 -> Terminator16/1
  Read Parameter23/2 -> Terminator17/1
  Read Parameter24/2 -> Terminator18/1
  Read Parameter28/2 -> Terminator19/1
  Read Parameter29/2 -> Terminator20/1
  Read Parameter11/1 -> Bus Creator3/8  "L2_ZZ"
  Read Parameter14/1 -> Bus Creator3/7  "L2_YY"
  Read Parameter13/1 -> Bus Creator3/6  "L2_XX"
  Read Parameter12/1 -> Bus Creator3/5  "L2_MASS"
  Read Parameter10/1 -> Bus Creator3/4  "L1_ZZ"
  Read Parameter9/1 -> Bus Creator3/3  "L1_YY"
  Read Parameter8/1 -> Bus Creator3/2  "L1_XX"
  Read Parameter2/1 -> Bus Creator3/1  "L1_MASS"
  Read Parameter2/2 -> Terminator21/1
  Read Parameter8/2 -> Terminator22/1
  Read Parameter9/2 -> Terminator23/1
  Read Parameter10/2 -> Terminator24/1
  Read Parameter12/2 -> Terminator25/1
  Read Parameter13/2 -> Terminator26/1
  Read Parameter14/2 -> Terminator27/1
  Read Parameter11/2 -> Terminator28/1
  Bus Creator3/1 -> [UAM_LINKS_DATA]  "Parameters"
  [UAM_LINKS_DATA] -> Bus Creator/4  "UAM_LINK_DATA"
  [ESO_OBSERVER] -> Bus Creator/5  "ESO_OBSERVER"
  Bus Creator4/1 -> [ESO_OBSERVER]
  Read Parameter30/2 -> Terminator30/1
  Read Parameter4/2 -> Terminator29/1
  Read Parameter31/2 -> Terminator31/1
  Read Parameter32/2 -> Terminator32/1
  Read Parameter35/2 -> Terminator33/1
  Read Parameter33/2 -> Terminator34/1
  Read Parameter34/2 -> Terminator35/1
  Read Parameter37/2 -> Terminator37/1
  Read Parameter36/2 -> Terminator36/1
  Read Parameter41/2 -> Terminator43/1
  Read Parameter48/2 -> Terminator49/1
  Read Parameter64/2 -> Terminator56/1
  Read Parameter93/2 -> Terminator83/1
  Read Parameter46/2 -> Terminator38/1
  Read Parameter38/2 -> Terminator39/1
  Read Parameter39/2 -> Terminator40/1
  Read Parameter40/2 -> Terminator41/1
  Read Parameter43/2 -> Terminator42/1
  Read Parameter42/2 -> Terminator44/1
  Read Parameter45/2 -> Terminator46/1
  Read Parameter44/2 -> Terminator45/1
  Read Parameter55/2 -> Terminator47/1
  Read Parameter47/2 -> Terminator48/1
  Read Parameter49/2 -> Terminator50/1
  Read Parameter52/2 -> Terminator51/1
  Read Parameter50/2 -> Terminator52/1
  Read Parameter51/2 -> Terminator53/1
  Read Parameter54/2 -> Terminator55/1
  Read Parameter53/2 -> Terminator54/1
  Read Parameter56/2 -> Terminator57/1
  Read Parameter57/2 -> Terminator58/1
  Read Parameter58/2 -> Terminator59/1
  Read Parameter61/2 -> Terminator60/1
  Read Parameter59/2 -> Terminator61/1
  Read Parameter60/2 -> Terminator62/1
  Read Parameter63/2 -> Terminator64/1
  Read Parameter62/2 -> Terminator63/1
  Read Parameter73/2 -> Terminator65/1
  Read Parameter65/2 -> Terminator66/1
  Read Parameter66/2 -> Terminator67/1
  Read Parameter67/2 -> Terminator68/1
  Read Parameter70/2 -> Terminator69/1
  Read Parameter68/2 -> Terminator70/1
  Read Parameter69/2 -> Terminator71/1
  Read Parameter72/2 -> Terminator73/1
  Read Parameter71/2 -> Terminator72/1
  Read Parameter82/2 -> Terminator74/1
  Read Parameter74/2 -> Terminator75/1
  Read Parameter75/2 -> Terminator76/1
  Read Parameter76/2 -> Terminator77/1
  Read Parameter79/2 -> Terminator78/1
  Read Parameter77/2 -> Terminator79/1
  Read Parameter78/2 -> Terminator80/1
  Read Parameter81/2 -> Terminator82/1
  Read Parameter80/2 -> Terminator81/1
  Read Parameter83/2 -> Terminator84/1
  Read Parameter84/2 -> Terminator85/1
  Read Parameter85/2 -> Terminator86/1
  Read Parameter88/2 -> Terminator87/1
  Read Parameter86/2 -> Terminator88/1
  Read Parameter87/2 -> Terminator89/1
  Read Parameter90/2 -> Terminator91/1
  Read Parameter100/2 -> Terminator92/1
  Read Parameter91/2 -> Terminator93/1
  Read Parameter92/2 -> Terminator94/1
  Read Parameter94/2 -> Terminator95/1
  Read Parameter97/2 -> Terminator96/1
  Read Parameter95/2 -> Terminator97/1
  Read Parameter96/2 -> Terminator98/1
  Read Parameter99/2 -> Terminator100/1
  Read Parameter98/2 -> Terminator99/1
  Read Parameter116/2 -> Terminator111/1
  Read Parameter107/1 -> Bus Creator5/9  "UAM_ROLL_P"
  Read Parameter106/2 -> Terminator101/1
  Read Parameter109/1 -> Bus Creator5/12  "UAM_PITCH_D"
  Read Parameter114/1 -> Bus Creator5/8  "UAM_L_ONE_D"
  Bus Creator5/1 -> Goto9/1
  Read Parameter110/2 -> Terminator108/1
  Read Parameter103/2 -> Terminator114/1
  Read Parameter112/2 -> Terminator105/1
  Read Parameter104/2 -> Terminator115/1
  Read Parameter113/2 -> Terminator102/1
  Read Parameter115/2 -> Terminator110/1
  Read Parameter114/2 -> Terminator103/1
  Read Parameter105/2 -> Terminator116/1
  Read Parameter102/1 -> Bus Creator5/1  "UAM_X_P"
  Read Parameter115/1 -> Bus Creator5/15  "UAM_L_TWO_P"
  Read Parameter117/2 -> Terminator113/1
  Read Parameter116/1 -> Bus Creator5/16  "UAM_L_TWO_D"
  Read Parameter107/2 -> Terminator104/1
  Read Parameter109/2 -> Terminator107/1
  Read Parameter111/1 -> Bus Creator5/14  "UAM_YAW_D"
  Read Parameter117/1 -> Bus Creator5/2  "UAM_X_D"
  Read Parameter105/1 -> Bus Creator5/5  "UAM_Z_P"
  Read Parameter104/1 -> Bus Creator5/4  "UAM_Y_D"
  Read Parameter106/1 -> Bus Creator5/6  "UAM_Z_D"
  Read Parameter108/1 -> Bus Creator5/11  "UAM_PITCH_P"
  Read Parameter102/2 -> Terminator112/1
  Read Parameter111/2 -> Terminator109/1
  Read Parameter108/2 -> Terminator106/1
  Read Parameter103/1 -> Bus Creator5/3  "UAM_Y_P"
  Read Parameter110/1 -> Bus Creator5/13  "UAM_YAW_P"
  Read Parameter113/1 -> Bus Creator5/7  "UAM_L_ONE_P"
  Read Parameter112/1 -> Bus Creator5/10  "UAM_ROLL_D"
  Bus Creator2/1 -> [PD_CTRL]
  Mux1/1 -> Bus Creator2/2  "Kd"
  Mux/1 -> Bus Creator2/1  "Kp"
  Read Parameter3/1 -> Mux1/1  "UAM_X_D"
  Read Parameter17/1 -> Mux1/2  "UAM_Y_D"
  Read Parameter19/1 -> Mux1/3  "UAM_Z_D"
  Read Parameter25/1 -> Mux1/4  "UAM_ROLL_D"
  Read Parameter22/1 -> Mux1/5  "UAM_PITCH_D"
  Read Parameter24/1 -> Mux1/6  "UAM_YAW_D"
  Read Parameter27/1 -> Mux1/7  "UAM_L_ONE_D"
  Read Parameter29/1 -> Mux1/8  "UAM_L_TWO_D"
  Read Parameter15/1 -> Mux/1  "UAM_X_P"
  Read Parameter16/1 -> Mux/2  "UAM_Y_P"
  Read Parameter18/1 -> Mux/3  "UAM_Z_P"
  Read Parameter20/1 -> Mux/4  "UAM_ROLL_P"
  Read Parameter21/1 -> Mux/5  "UAM_PITCH_P"
  Read Parameter23/1 -> Mux/6  "UAM_YAW_P"
  Read Parameter26/1 -> Mux/7  "UAM_L_ONE_P"
  Read Parameter28/1 -> Mux/8  "UAM_L_TWO_P"
  Read Parameter180/1 -> Bus Creator6/62  "L1_ALPHA"
  Read Parameter180/2 -> Terminator180/1
  Read Parameter161/1 -> Bus Creator6/45  "PITCH_BETA"
  Read Parameter176/2 -> Terminator177/1
  Read Parameter152/1 -> Bus Creator6/36  "ROLL_BETA"
  Read Parameter125/1 -> Bus Creator6/9  "X_BETA"
  Read Parameter131/2 -> Terminator132/1
  Read Parameter162/1 -> Bus Creator6/44  "PITCH_ALPHA"
  Read Parameter145/2 -> Terminator136/1
  Read Parameter126/1 -> Bus Creator6/8  "X_ALPHA"
  Read Parameter123/1 -> Bus Creator6/7  "X_MU3"
  Read Parameter157/2 -> Terminator157/1
  Read Parameter187/2 -> Terminator185/1
  Read Parameter181/1 -> Bus Creator6/65  "L2_E2"
  Read Parameter182/2 -> Terminator183/1
  Read Parameter163/1 -> Bus Creator6/37  "PITCH_E1"
  Read Parameter175/2 -> Terminator175/1
  Read Parameter147/2 -> Terminator147/1
  Read Parameter119/2 -> Terminator119/1
  Read Parameter141/1 -> Bus Creator6/25  "Z_MU3"
  Read Parameter150/2 -> Terminator151/1
  Read Parameter125/2 -> Terminator125/1
  Read Parameter129/2 -> Terminator118/1
  Read Parameter184/1 -> Bus Creator6/67  "L2_E4"
  Read Parameter174/1 -> Bus Creator6/57  "L1_E3"
  Read Parameter183/2 -> Terminator172/1
  Read Parameter129/1 -> Bus Creator6/1  "X_E1"
  Read Parameter149/2 -> Terminator150/1
  Read Parameter127/1 -> Bus Creator6/11  "Y_E2"
  Read Parameter132/2 -> Terminator133/1
  Bus Creator6/1 -> Goto10/1
  Read Parameter169/2 -> Terminator167/1
  Read Parameter154/2 -> Terminator145/1
  Read Parameter138/2 -> Terminator138/1
  Read Parameter185/2 -> Terminator186/1
  Read Parameter160/2 -> Terminator158/1
  Read Parameter166/2 -> Terminator166/1
  Read Parameter179/2 -> Terminator179/1
  Read Parameter173/2 -> Terminator173/1
  Read Parameter183/1 -> Bus Creator6/55  "L1_E1"
  Read Parameter148/2 -> Terminator148/1
  Read Parameter186/2 -> Terminator187/1
  Read Parameter166/1 -> Bus Creator6/49  "YAW_E4"
  Read Parameter181/2 -> Terminator182/1
  Read Parameter173/1 -> Bus Creator6/56  "L1_E2"
  Read Parameter143/1 -> Bus Creator6/27  "Z_BETA"
  Read Parameter149/1 -> Bus Creator6/33  "ROLL_MU2"
  Read Parameter147/1 -> Bus Creator6/30  "ROLL_E3"
  Read Parameter158/1 -> Bus Creator6/42  "PITCH_MU2"
  Read Parameter156/1 -> Bus Creator6/39  "PITCH_E3"
  Read Parameter157/1 -> Bus Creator6/40  "PITCH_E4"
  Read Parameter138/1 -> Bus Creator6/21  "Z_E3"
  Read Parameter167/2 -> Terminator168/1
  Read Parameter140/1 -> Bus Creator6/24  "Z_MU2"
  Read Parameter186/1 -> Bus Creator6/70  "L2_MU3"
  Read Parameter168/1 -> Bus Creator6/52  "YAW_MU3"
  Read Parameter135/2 -> Terminator135/1
  Read Parameter175/1 -> Bus Creator6/58  "L1_E4"
  Read Parameter140/2 -> Terminator141/1
  Read Parameter139/2 -> Terminator139/1
  Read Parameter134/2 -> Terminator134/1
  Read Parameter128/1 -> Bus Creator6/12  "Y_E3"
  Read Parameter128/2 -> Terminator129/1
  Read Parameter146/1 -> Bus Creator6/29  "ROLL_E2"
  Read Parameter159/1 -> Bus Creator6/43  "PITCH_MU3"
  Read Parameter118/2 -> Terminator181/1
  Read Parameter153/2 -> Terminator153/1
  Read Parameter187/1 -> Bus Creator6/68  "L2_MU1"
  Read Parameter145/1 -> Bus Creator6/19  "Z_E1"
  Read Parameter176/1 -> Bus Creator6/60  "L1_MU2"
  Read Parameter161/2 -> Terminator161/1
  Read Parameter165/2 -> Terminator165/1
  Read Parameter127/2 -> Terminator128/1
  Read Parameter152/2 -> Terminator152/1
  Read Parameter154/1 -> Bus Creator6/28  "ROLL_E1"
  Read Parameter174/2 -> Terminator174/1
  Read Parameter124/1 -> Bus Creator6/5  "X_MU1"
  Read Parameter146/2 -> Terminator146/1
  Read Parameter142/1 -> Bus Creator6/23  "Z_MU1"
  Read Parameter163/2 -> Terminator154/1
  Read Parameter130/2 -> Terminator130/1
  Read Parameter136/1 -> Bus Creator6/10  "Y_E1"
  Read Parameter136/2 -> Terminator127/1
  Read Parameter178/2 -> Terminator176/1
  Read Parameter132/1 -> Bus Creator6/16  "Y_MU3"
  Read Parameter188/1 -> Bus Creator6/72  "L2_BETA"
  Read Parameter160/1 -> Bus Creator6/41  "PITCH_MU1"
  Read Parameter133/1 -> Bus Creator6/14  "Y_MU1"
  Read Parameter170/2 -> Terminator170/1
  Read Parameter121/1 -> Bus Creator6/4  "X_E4"
  Read Parameter159/2 -> Terminator160/1
  Read Parameter179/1 -> Bus Creator6/63  "L1_BETA"
  Read Parameter182/1 -> Bus Creator6/66  "L2_E3"
  Read Parameter156/2 -> Terminator156/1
  Read Parameter139/1 -> Bus Creator6/22  "Z_E4"
  Read Parameter184/2 -> Terminator184/1
  Read Parameter188/2 -> Terminator188/1
  Read Parameter171/2 -> Terminator171/1
  Read Parameter155/1 -> Bus Creator6/38  "PITCH_E2"
  Read Parameter169/1 -> Bus Creator6/50  "YAW_MU1"
  Read Parameter148/1 -> Bus Creator6/31  "ROLL_E4"
  Read Parameter143/2 -> Terminator143/1
  Read Parameter153/1 -> Bus Creator6/35  "ROLL_ALPHA"
  Read Parameter142/2 -> Terminator140/1
  Read Parameter164/2 -> Terminator164/1
  Read Parameter177/2 -> Terminator178/1
  Read Parameter131/1 -> Bus Creator6/15  "Y_MU2"
  Read Parameter137/2 -> Terminator137/1
  Read Parameter172/2 -> Terminator163/1
  Read Parameter164/1 -> Bus Creator6/47  "YAW_E2"
  Read Parameter123/2 -> Terminator124/1
  Read Parameter172/1 -> Bus Creator6/46  "YAW_E1"
  Read Parameter122/2 -> Terminator123/1
  Read Parameter137/1 -> Bus Creator6/20  "Z_E2"
  Read Parameter119/1 -> Bus Creator6/2  "X_E2"
  Read Parameter185/1 -> Bus Creator6/69  "L2_MU2"
  Read Parameter141/2 -> Terminator142/1
  Read Parameter122/1 -> Bus Creator6/6  "X_MU2"
  Read Parameter133/2 -> Terminator131/1
  Read Parameter155/2 -> Terminator155/1
  Read Parameter144/1 -> Bus Creator6/26  "Z_ALPHA"
  Read Parameter151/1 -> Bus Creator6/32  "ROLL_MU1"
  Read Parameter167/1 -> Bus Creator6/51  "YAW_MU2"
  Read Parameter162/2 -> Terminator162/1
  Read Parameter158/2 -> Terminator159/1
  Read Parameter177/1 -> Bus Creator6/61  "L1_MU3"
  Read Parameter150/1 -> Bus Creator6/34  "ROLL_MU3"
  Read Parameter189/1 -> Bus Creator6/71  "L2_ALPHA"
  Read Parameter171/1 -> Bus Creator6/53  "YAW_ALPHA"
  Read Parameter120/2 -> Terminator120/1
  Read Parameter120/1 -> Bus Creator6/3  "X_E3"
  Read Parameter126/2 -> Terminator126/1
  Read Parameter189/2 -> Terminator117/1
  Read Parameter121/2 -> Terminator121/1
  Read Parameter134/1 -> Bus Creator6/18  "Y_BETA"
  Read Parameter178/1 -> Bus Creator6/59  "L1_MU1"
  Read Parameter124/2 -> Terminator122/1
  Read Parameter144/2 -> Terminator144/1
  Read Parameter151/2 -> Terminator149/1
  Read Parameter118/1 -> Bus Creator6/64  "L2_E1"
  Read Parameter170/1 -> Bus Creator6/54  "YAW_BETA"
  Read Parameter168/2 -> Terminator169/1
  Read Parameter130/1 -> Bus Creator6/13  "Y_E4"
  Read Parameter165/1 -> Bus Creator6/48  "YAW_E3"
  Read Parameter135/1 -> Bus Creator6/17  "Y_ALPHA"
  Read Parameter89/2 -> Terminator90/1
  Read Parameter4/1 -> Mux2/1  "X_E1"
  Read Parameter46/1 -> Mux2/2  "Y_E1"
  Read Parameter55/1 -> Mux2/3  "Z_E1"
  Read Parameter64/1 -> Mux2/4  "ROLL_E1"
  Read Parameter73/1 -> Mux2/5  "PITCH_E1"
  Read Parameter82/1 -> Mux2/6  "YAW_E1"
  Read Parameter93/1 -> Mux2/7  "L1_E1"
  Read Parameter100/1 -> Mux2/8  "L2_E1"
  Read Parameter30/1 -> Mux3/1  "X_E2"
  Read Parameter38/1 -> Mux3/2  "Y_E2"
  Read Parameter47/1 -> Mux3/3  "Z_E2"
  Read Parameter56/1 -> Mux3/4  "ROLL_E2"
  Read Parameter91/1 -> Mux3/8  "L2_E2"
  Read Parameter83/1 -> Mux3/7  "L1_E2"
  Read Parameter65/1 -> Mux3/5  "PITCH_E2"
  Read Parameter74/1 -> Mux3/6  "YAW_E2"
  Read Parameter31/1 -> Mux4/1  "X_E3"
  Read Parameter39/1 -> Mux4/2  "Y_E3"
  Read Parameter48/1 -> Mux4/3  "Z_E3"
  Read Parameter57/1 -> Mux4/4  "ROLL_E3"
  Read Parameter66/1 -> Mux4/5  "PITCH_E3"
  Read Parameter75/1 -> Mux4/6  "YAW_E3"
  Read Parameter84/1 -> Mux4/7  "L1_E3"
  Read Parameter92/1 -> Mux4/8  "L2_E3"
  Read Parameter32/1 -> Mux5/1  "X_E4"
  Read Parameter40/1 -> Mux5/2  "Y_E4"
  Read Parameter49/1 -> Mux5/3  "Z_E4"
  Read Parameter58/1 -> Mux5/4  "ROLL_E4"
  Read Parameter67/1 -> Mux5/5  "PITCH_E4"
  Read Parameter76/1 -> Mux5/6  "YAW_E4"
  Read Parameter85/1 -> Mux5/7  "L1_E4"
  Read Parameter94/1 -> Mux5/8  "L2_E4"
  Read Parameter35/1 -> Mux6/1  "X_MU1"
  Read Parameter43/1 -> Mux6/2  "Y_MU1"
  Read Parameter52/1 -> Mux6/3  "Z_MU1"
  Read Parameter61/1 -> Mux6/4  "ROLL_MU1"
  Read Parameter70/1 -> Mux6/5  "PITCH_MU1"
  Read Parameter79/1 -> Mux6/6  "YAW_MU1"
  Read Parameter88/1 -> Mux6/7  "L1_MU1"
  Read Parameter97/1 -> Mux6/8  "L2_MU1"
  Read Parameter33/1 -> Mux7/1  "X_MU2"
  Read Parameter41/1 -> Mux7/2  "Y_MU2"
  Read Parameter50/1 -> Mux7/3  "Z_MU2"
  Read Parameter59/1 -> Mux7/4  "ROLL_MU2"
  Read Parameter68/1 -> Mux7/5  "PITCH_MU2"
  Read Parameter77/1 -> Mux7/6  "YAW_MU2"
  Read Parameter86/1 -> Mux7/7  "L1_MU2"
  Read Parameter95/1 -> Mux7/8  "L2_MU2"
  Read Parameter34/1 -> Mux8/1  "X_MU3"
  Read Parameter42/1 -> Mux8/2  "Y_MU3"
  Read Parameter51/1 -> Mux8/3  "Z_MU3"
  Read Parameter60/1 -> Mux8/4  "ROLL_MU3"
  Read Parameter69/1 -> Mux8/5  "PITCH_MU3"
  Read Parameter78/1 -> Mux8/6  "YAW_MU3"
  Read Parameter87/1 -> Mux8/7  "L1_MU3"
  Read Parameter96/1 -> Mux8/8  "L2_MU3"
  Read Parameter37/1 -> Mux9/1  "X_ALPHA"
  Read Parameter45/1 -> Mux9/2  "Y_ALPHA"
  Read Parameter54/1 -> Mux9/3  "Z_ALPHA"
  Read Parameter63/1 -> Mux9/4  "ROLL_ALPHA"
  Read Parameter72/1 -> Mux9/5  "PITCH_ALPHA"
  Read Parameter81/1 -> Mux9/6  "YAW_ALPHA"
  Read Parameter90/1 -> Mux9/7  "L1_ALPHA"
  Read Parameter99/1 -> Mux9/8  "L2_ALPHA"
  Read Parameter36/1 -> Mux10/1  "X_BETA"
  Read Parameter44/1 -> Mux10/2  "Y_BETA"
  Read Parameter53/1 -> Mux10/3  "Z_BETA"
  Read Parameter62/1 -> Mux10/4  "ROLL_BETA"
  Read Parameter71/1 -> Mux10/5  "PITCH_BETA"
  Read Parameter80/1 -> Mux10/6  "YAW_BETA"
  Read Parameter89/1 -> Mux10/7  "L1_BETA"
  Read Parameter98/1 -> Mux10/8  "L2_BETA"
  Mux2/1 -> Bus Creator4/1  "E1"
  Mux3/1 -> Bus Creator4/2  "E2"
  Mux4/1 -> Bus Creator4/3  "E3"
  Mux5/1 -> Bus Creator4/4  "E4"
  Mux6/1 -> Bus Creator4/5  "MU1"
  Mux7/1 -> Bus Creator4/6  "MU2"
  Mux8/1 -> Bus Creator4/7  "MU3"
  Mux9/1 -> Bus Creator4/8  "ALPHA"
  Mux10/1 -> Bus Creator4/9  "BETA"
